simulink model "LongitudinalDoublet"  (R2021b)
settings: Solver=VariableStepAuto  StartTime=0.0  StopTime=60  RelTol=1e-3
libraries: LPVBlockLibrary x4
settings Model: Creator=jihoo  LastModifiedBy=jihoo

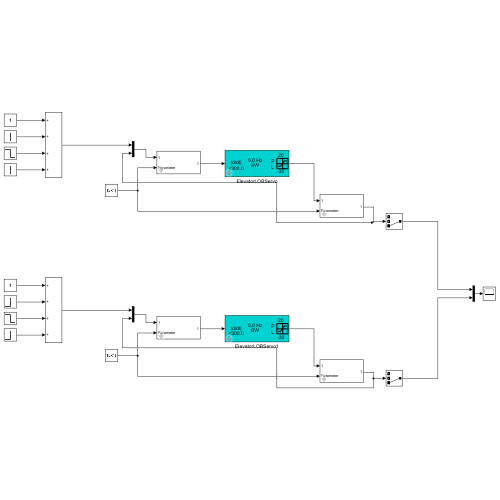
[thumbnail: Simulink's stored preview of the top-level diagram]
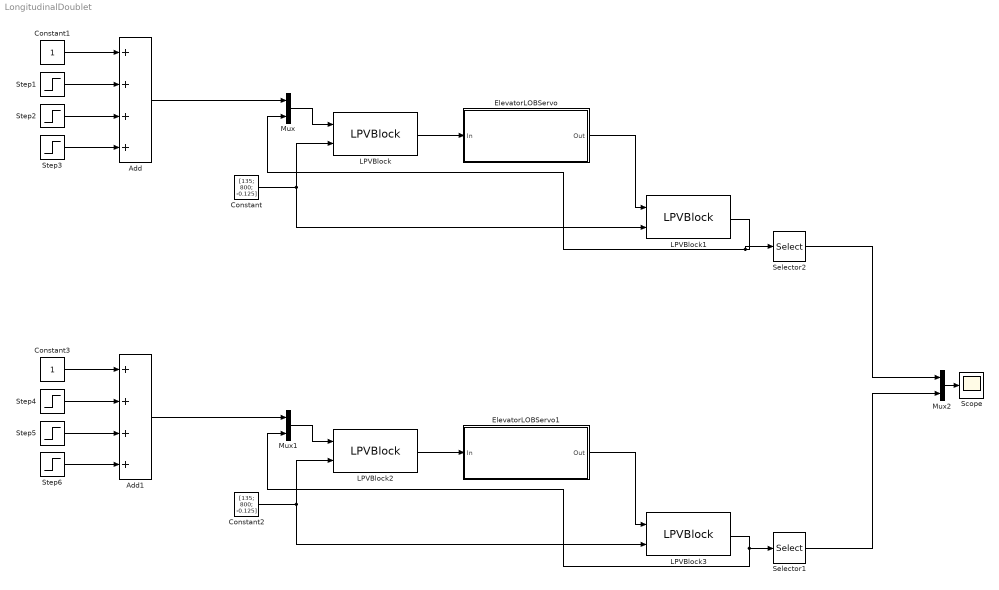
== system LongitudinalDoublet ==
  Add : Sum  Inputs=++++
  Add1 : Sum  Inputs=++++
  Constant : Constant  Value=[135; 800; -0.125]
  Constant1 : Constant
  Constant2 : Constant  Value=[135; 800; -0.125]
  Constant3 : Constant
  ElevatorLOBServo : Subsystem  mask(Rate and Position Limited Servo){freq=5, RL=300, POS_hi=20, POS_lo=-30, Bias=0}
      mask prompts: freq "Bandwidth, Hz"; RL "Rate Limit:"; POS_hi "Position Limit High:"; POS_lo "Position Limit Low:"; Bias "Bias Value:"
      mask help:
      | First order transfer function: w/(s+w), with rate and position limits
      | and output bias level.
      mask Display:
      | text(.48,.55,sprintf('%3.1f Hz\nBW',freq),'horizontalAlignment','center');
      | 
      | text(0.18,0.45,sprintf('|d/dt|\n<%0.1f',RL),'horizontalAlignment','center');
      | 
      | text(0.88,0.85,num2str(POS_hi),'horizontalAlignment', 'center');
      | text(0.88,0.2,num2str(POS_lo),'horizontalAlignment', 'center');
      | text(0.73,0.5,'P\nL');
      | 
      | 
      | plot([0.83 0.87 0.93 0.97],[0.4 0.4 0.6 0.6]);
      | plot([0.81 0.99],[0.5 0.5]);
      | plot([0.9 0.9],[0.3 0.7]);
      | plot([0.81 0.99 0.99 0.81 0.81],[0.3 0.3 0.7 0.7 0.3]);
  ElevatorLOBServo1 : Subsystem  mask(Rate and Position Limited Servo){freq=5, RL=300, POS_hi=20, POS_lo=-30, Bias=0}
      mask prompts: freq "Bandwidth, Hz"; RL "Rate Limit:"; POS_hi "Position Limit High:"; POS_lo "Position Limit Low:"; Bias "Bias Value:"
      mask help:
      | First order transfer function: w/(s+w), with rate and position limits
      | and output bias level.
      mask Display:
      | text(.48,.55,sprintf('%3.1f Hz\nBW',freq),'horizontalAlignment','center');
      | 
      | text(0.18,0.45,sprintf('|d/dt|\n<%0.1f',RL),'horizontalAlignment','center');
      | 
      | text(0.88,0.85,num2str(POS_hi),'horizontalAlignment', 'center');
      | text(0.88,0.2,num2str(POS_lo),'horizontalAlignment', 'center');
      | text(0.73,0.5,'P\nL');
      | 
      | 
      | plot([0.83 0.87 0.93 0.97],[0.4 0.4 0.6 0.6]);
      | plot([0.81 0.99],[0.5 0.5]);
      | plot([0.9 0.9],[0.3 0.7]);
      | plot([0.81 0.99 0.99 0.81 0.81],[0.3 0.3 0.7 0.7 0.3]);
  LPVBlock : LPVBlockLibrary/LPVBlock  sys=K_lon_lpv  plist={'rho1_tas_param';'rho2_alt_param';'rho3_mor_param'}  x0=0
      settings: SourceProductName=LPVTools Blocks
  LPVBlock1 : LPVBlockLibrary/LPVBlock  sys=P_lon  plist={'rho1_tas_param';'rho2_alt_param';'rho3_mor_param'}  x0=0
      settings: SourceProductName=LPVTools Blocks
  LPVBlock2 : LPVBlockLibrary/LPVBlock  sys=K_lon_hinf  plist={'rho1_tas_param';'rho2_alt_param';'rho3_mor_param'}  x0=0
      settings: SourceProductName=LPVTools Blocks
  LPVBlock3 : LPVBlockLibrary/LPVBlock  sys=P_lon  plist={'rho1_tas_param';'rho2_alt_param';'rho3_mor_param'}  x0=0
      settings: SourceProductName=LPVTools Blocks
  Mux : Mux  Inputs=2
  Mux1 : Mux  Inputs=2
  Mux2 : Mux  Inputs=2
  Scope : Scope
  Selector1 : Selector  InputPortWidth=3  IndexOptions=Index vector (dialog)  Indices=3  OutputSizes=1
  Selector2 : Selector  InputPortWidth=3  IndexOptions=Index vector (dialog)  Indices=3  OutputSizes=1
  Step1 : Step  SampleTime=0
  Step2 : Step  Time=5  After=-2  SampleTime=0
  Step3 : Step  Time=9  SampleTime=0
  Step4 : Step  SampleTime=0
  Step5 : Step  Time=5  After=-2  SampleTime=0
  Step6 : Step  Time=9  SampleTime=0
  wires:
  LPVBlock/1 -> ElevatorLOBServo/1(In)
  Constant/1 -> LPVBlock1/2, LPVBlock/2
  Add/1 -> Mux/1
  LPVBlock1/1 -> Selector2/1, Mux/2
  Mux/1 -> LPVBlock/1
  Step3/1 -> Add/4
  Step1/1 -> Add/2
  Constant1/1 -> Add/1
  Step2/1 -> Add/3
  ElevatorLOBServo/1(Out) -> LPVBlock1/1
  ElevatorLOBServo1/1(Out) -> LPVBlock3/1
  Step5/1 -> Add1/3
  Constant3/1 -> Add1/1
  Step4/1 -> Add1/2
  Step6/1 -> Add1/4
  Mux1/1 -> LPVBlock2/1
  LPVBlock3/1 -> Selector1/1, Mux1/2
  Add1/1 -> Mux1/1
  Constant2/1 -> LPVBlock2/2, LPVBlock3/2
  LPVBlock2/1 -> ElevatorLOBServo1/1(In)
  Selector1/1 -> Mux2/2
  Mux2/1 -> Scope/1
  Selector2/1 -> Mux2/1

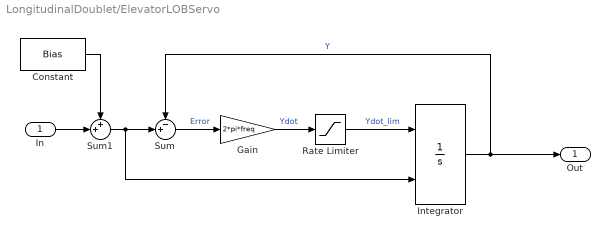
== system LongitudinalDoublet/ElevatorLOBServo ==
  In : Inport
  Constant : Constant  Value=Bias
  Gain : Gain  Gain=2*pi*freq  SaturateOnIntegerOverflow=on  OutDataTypeStr=Inherit: Same as input  ParamDataTypeStr=Inherit: Same as input
  Integrator : Integrator  InitialConditionSource=external  LimitOutput=on  UpperSaturationLimit=POS_hi  LowerSaturationLimit=POS_lo  IgnoreLimit=on
  Rate Limiter : Saturate  UpperLimit=RL  LowerLimit=-RL
  Sum : Sum  Inputs=-+|  InputSameDT=on  SaturateOnIntegerOverflow=on  OutDataTypeStr=Inherit: Same as first input
  Sum1 : Sum  Inputs=++|  InputSameDT=on  SaturateOnIntegerOverflow=on  OutDataTypeStr=Inherit: Same as first input
  Out : Outport  PortDimensions=1
  wires:
  Constant/1 -> Sum1/1
  Sum1/1 -> Integrator/2, Sum/2
  In/1 -> Sum1/2
  Rate Limiter/1 -> Integrator/1  "Ydot_lim"
  Integrator/1 -> Out/1, Sum/1  "Y"
  Sum/1 -> Gain/1  "Error"
  Gain/1 -> Rate Limiter/1  "Ydot"

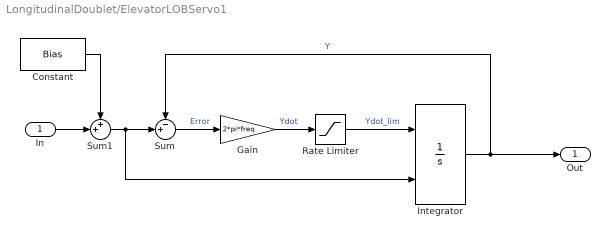
== system LongitudinalDoublet/ElevatorLOBServo1 ==
  In : Inport
  Constant : Constant  Value=Bias
  Gain : Gain  Gain=2*pi*freq  SaturateOnIntegerOverflow=on  OutDataTypeStr=Inherit: Same as input  ParamDataTypeStr=Inherit: Same as input
  Integrator : Integrator  InitialConditionSource=external  LimitOutput=on  UpperSaturationLimit=POS_hi  LowerSaturationLimit=POS_lo  IgnoreLimit=on
  Rate Limiter : Saturate  UpperLimit=RL  LowerLimit=-RL
  Sum : Sum  Inputs=-+|  InputSameDT=on  SaturateOnIntegerOverflow=on  OutDataTypeStr=Inherit: Same as first input
  Sum1 : Sum  Inputs=++|  InputSameDT=on  SaturateOnIntegerOverflow=on  OutDataTypeStr=Inherit: Same as first input
  Out : Outport  PortDimensions=1
  wires:
  Gain/1 -> Rate Limiter/1  "Ydot"
  Sum/1 -> Gain/1  "Error"
  Integrator/1 -> Sum/1, Out/1  "Y"
  Rate Limiter/1 -> Integrator/1  "Ydot_lim"
  In/1 -> Sum1/2
  Sum1/1 -> Sum/2, Integrator/2
  Constant/1 -> Sum1/1
